simulink model "quad_sim"  (R2024b)
settings: Solver=ode45  StartTime=0.0  StopTime=P.Tsim  MaxStep=1e-3  RelTol=1e-3
InitFcn:
  | if ~exist('P','var'), quad_params; end
values from neighbouring files (symbols this model uses):
  P = struct()    [quad_params.m]
settings Model: Creator=wassim Toukebri  LastModifiedBy=wassim Toukebri

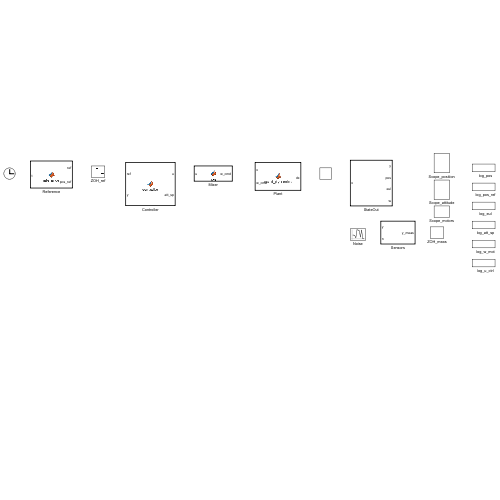
[thumbnail: Simulink's stored preview of the top-level diagram]
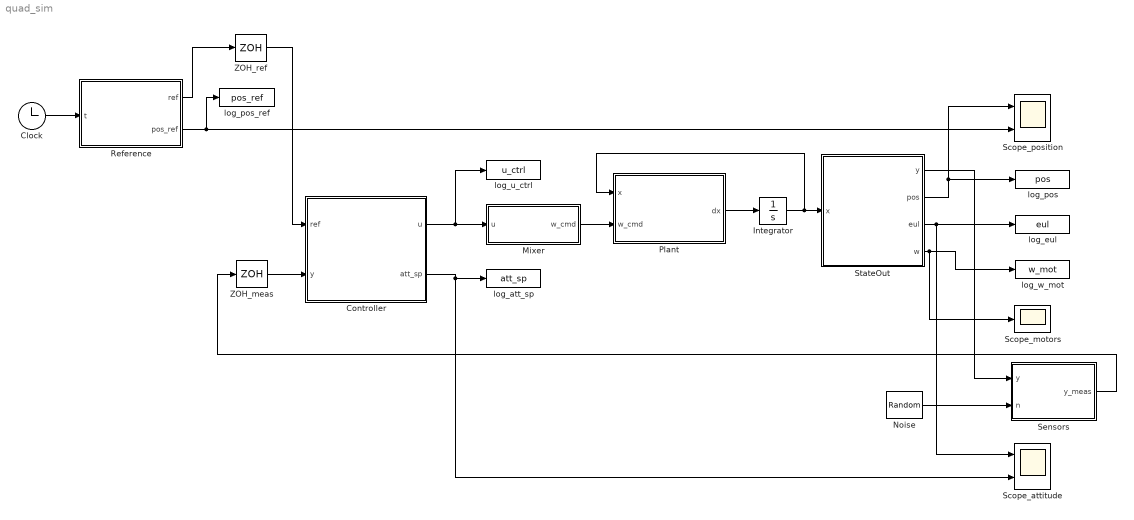
== system quad_sim ==
  Clock : Clock
  Controller : MATLAB Function  TreatAsAtomicUnit=on
  Integrator : Integrator  InitialCondition=P.x0
  Mixer : MATLAB Function  TreatAsAtomicUnit=on
  Noise : RandomNumber  Mean=zeros(1,12)  Variance=P.sens.enable*P.sens.std.^2  Seed=1:12  SampleTime=P.Ts
  Plant : MATLAB Function  TreatAsAtomicUnit=on
  Reference : MATLAB Function  TreatAsAtomicUnit=on
  Scope_attitude : Scope  NumInputPorts=2
  Scope_motors : Scope
  Scope_position : Scope  NumInputPorts=2
  Sensors : MATLAB Function  TreatAsAtomicUnit=on
  StateOut : MATLAB Function  TreatAsAtomicUnit=on
  ZOH_meas : ZeroOrderHold  SampleTime=P.Ts
  ZOH_ref : ZeroOrderHold  SampleTime=P.Ts
  log_att_sp : ToWorkspace  VariableName=att_sp  SaveFormat=Timeseries  SampleTime=-1
  log_eul : ToWorkspace  VariableName=eul  SaveFormat=Timeseries  SampleTime=-1
  log_pos : ToWorkspace  VariableName=pos  SaveFormat=Timeseries  SampleTime=-1
  log_pos_ref : ToWorkspace  VariableName=pos_ref  SaveFormat=Timeseries  SampleTime=-1
  log_u_ctrl : ToWorkspace  VariableName=u_ctrl  SaveFormat=Timeseries  SampleTime=-1
  log_w_mot : ToWorkspace  VariableName=w_mot  SaveFormat=Timeseries  SampleTime=-1
  wires:
  Controller/1(u) -> Mixer/1(u), log_u_ctrl/1
  ZOH_meas/1 -> Controller/2(y)
  Clock/1 -> Reference/1(t)
  StateOut/4(w) -> Scope_motors/1, log_w_mot/1
  ZOH_ref/1 -> Controller/1(ref)
  StateOut/1(y) -> Sensors/1(y)
  Reference/2(pos_ref) -> Scope_position/2, log_pos_ref/1
  Reference/1(ref) -> ZOH_ref/1
  Controller/2(att_sp) -> Scope_attitude/2, log_att_sp/1
  Mixer/1(w_cmd) -> Plant/2(w_cmd)
  Plant/1(dx) -> Integrator/1
  Integrator/1 -> StateOut/1(x), Plant/1(x)
  Noise/1 -> Sensors/2(n)
  StateOut/2(pos) -> Scope_position/1, log_pos/1
  StateOut/3(eul) -> Scope_attitude/1, log_eul/1
  Sensors/1(y_meas) -> ZOH_meas/1

== matlab function quad_sim/Controller ==
  data: ref input; u output; y input; att_sp output; P parameter
function [u, att_sp] = controller(ref, y, P)
% Cascaded flight controller, runs at P.Ts (discrete).
%   position -> tilt angles -> body rates -> torques ;  altitude -> thrust
% ref = [x y z psi phi theta],  y = measured [pos; vel; eul; omega]
% u   = [T; tau_x; tau_y; tau_z],  att_sp = [phi_sp; theta_sp; psi_sp]
persistent iz irate omega_prev dfilt zref_prev
if isempty(iz)
    iz = 0; irate = zeros(3,1); omega_prev = zeros(3,1); dfilt = zeros(3,1);
    zref_prev = 0;
end
Ts = P.Ts;  C = P.ctl;
pos = y(1:3); vel = y(4:6); eul = y(7:9); omega = y(10:12);

% ---------- disarmed on the ground: motors off, reset integrators
if ref(3) <= 0 && pos(3) < 0.05
    iz = 0; irate = zeros(3,1); dfilt = zeros(3,1); omega_prev = omega;
    zref_prev = ref(3);
    u = zeros(4,1);
    att_sp = [0; 0; ref(4)];
    return
end

% ---------- outer loop: position -> desired roll/pitch
if C.mode == 1
    e_p = ref(1:2) - pos(1:2);
    a_d = C.pos.Kp(:).*e_p - C.pos.Kd(:).*vel(1:2);
    a_d = min(max(a_d, -C.acc_max), C.acc_max);
    psi = eul(3);
    ax_b =  cos(psi)*a_d(1) + sin(psi)*a_d(2);   % rotate into yaw frame
    ay_b = -sin(psi)*a_d(1) + cos(psi)*a_d(2);
    theta_d = atan2(ax_b, P.g);
    phi_d   = atan2(-ay_b*cos(theta_d), P.g);
else
    phi_d   = ref(5);
    theta_d = ref(6);
end
phi_d   = min(max(phi_d,   -C.tilt_max), C.tilt_max);
theta_d = min(max(theta_d, -C.tilt_max), C.tilt_max);

% ---------- altitude loop -> collective thrust
vz_ref = (ref(3) - zref_prev)/Ts;               % climb-rate feed-forward
vz_ref = min(max(vz_ref, -C.vz_max), C.vz_max);  % (clipped so z steps don't spike)
zref_prev = ref(3);
ez = ref(3) - pos(3);
iz = min(max(iz + C.alt.Ki*ez*Ts, -C.alt.Imax), C.alt.Imax);
T  = P.m*P.g + C.alt.Kp*ez + C.alt.Kd*(vz_ref - vel(3)) + iz;
T  = T / max(cos(eul(1))*cos(eul(2)), 0.5);      % tilt compensation
T  = min(max(T, 0), C.T_max);

% ---------- attitude loop (P) -> rate setpoints
att_sp = [phi_d; theta_d; ref(4)];
e_att  = att_sp - eul;
e_att(3) = atan2(sin(e_att(3)), cos(e_att(3)));  % wrap yaw error
rate_sp = C.att.Kp(:).*e_att;
rate_sp = min(max(rate_sp, -C.rate_max(:)), C.rate_max(:));

% ---------- rate loop (PID, D on measurement, filtered)
e_r   = rate_sp - omega;
irate = min(max(irate + C.rate.Ki(:).*e_r*Ts, -C.rate.Imax(:)), C.rate.Imax(:));
d_raw = (omega - omega_prev)/Ts;
omega_prev = omega;
alpha = Ts/(Ts + 1/(2*pi*C.rate.dfc));
dfilt = dfilt + alpha*(d_raw - dfilt);
tau = C.rate.Kp(:).*e_r + irate - C.rate.Kd(:).*dfilt;

u = [T; tau];
end

== matlab function quad_sim/Reference ==
  data: t input; ref output; pos_ref output
function [ref, pos_ref] = reference(t)
% Mission profile.  ref = [x; y; z; psi; phi; theta]
% (phi/theta are only used when P.ctl.mode = 0, angle mode)
x = 0; y = 0; z = 0; psi = 0; phi = 0; theta = 0;
if t >= 1,  z   = min(1.5, 0.75*(t - 1)); end    % take-off ramp to 1.5 m
if t >= 6,  x   = 2;      end                    % move 2 m forward
if t >= 11, y   = 2;      end                    % move 2 m left
if t >= 16, psi = pi/2;   end                    % yaw 90 deg
if t >= 21, x = 0; y = 0; end                    % back above take-off point
if t >= 26, z   = max(0, 1.5 - 0.5*(t - 26)); end % landing ramp
ref     = [x; y; z; psi; phi; theta];
pos_ref = [x; y; z];
end

== matlab function quad_sim/Mixer ==
  data: u input; w_cmd output; P parameter
function w_cmd = mixer(u, P)
% Converts [T; tau_x; tau_y; tau_z] into the 4 motor speed commands.
% On the real board this is where you go to PWM / DShot values.
F = P.Ainv * u;              % thrust needed from each motor [N]
F = max(F, 0);               % props can't push down
w_cmd = sqrt(F / P.kf);
w_cmd = min(w_cmd, P.w_max);
end

== matlab function quad_sim/Plant ==
  data: x input; dx output; w_cmd input; P parameter
function dx = quad_dynamics(x, w_cmd, P)
% Quadcopter 6-DOF rigid body + first-order motors (Newton-Euler).
% x = [pos(3); vel(3); eul(3)=[phi theta psi]; omega(3)=[p q r]; w(4)]
% w_cmd = commanded motor speeds [rad/s]
vel   = x(4:6);
eul   = x(7:9);
omega = x(10:12);
w     = x(13:16);

% --- motors
w_c = min(max(w_cmd, 0), P.w_max);
dw  = (w_c - w) / P.tau_m;
F   = P.kf * w.^2;               % thrust of each motor
u   = P.A * F;                   % [T; tau_x; tau_y; tau_z]
T   = u(1);
tau = u(2:4);

% --- rotation body -> inertial (ZYX)
cph = cos(eul(1)); sph = sin(eul(1));
cth = cos(eul(2)); sth = sin(eul(2));
cps = cos(eul(3)); sps = sin(eul(3));
R = [cps*cth, cps*sth*sph - sps*cph, cps*sth*cph + sps*sph;
     sps*cth, sps*sth*sph + cps*cph, sps*sth*cph - cps*sph;
     -sth,    cth*sph,               cth*cph];

% --- translational dynamics
dpos = vel;
acc  = [0; 0; -P.g] + R*[0; 0; T]/P.m - (P.kd/P.m)*vel;

% --- rotational dynamics
Wm = [1, sph*sth/cth, cph*sth/cth;
      0, cph,         -sph;
      0, sph/cth,     cph/cth];
deul   = Wm * omega;
domega = P.J \ (tau - cross(omega, P.J*omega));

% --- simple ground contact (z = 0 plane)
if x(3) <= 0 && acc(3) <= 0
    dpos   = [0; 0; 0];
    acc    = -vel / 0.02;
    deul   = [0; 0; 0];
    domega = -omega / 0.02;
end

dx = [dpos; acc; deul; domega; dw];
end

== matlab function quad_sim/StateOut ==
  data: x input; y output; pos output; eul output; w output
function [y, pos, eul, w] = state_out(x)
% Splits the state vector into the signals that leave the plant.
y   = x(1:12);     % [pos; vel; eul; omega] -> goes to the sensors/controller
pos = x(1:3);
eul = x(7:9);
w   = x(13:16);    % motor speeds [rad/s]
end

== matlab function quad_sim/Sensors ==
  data: y input; y_meas output; n input
function y_meas = sensors(y, n)
% Measured state = true state + noise.  Replace with an IMU/baro/GPS model
% and a state estimator (complementary / Kalman filter) later.
y_meas = y + n(:);
end
